simulink model "fcn2A"  (Simulink 7.1)
settings: Solver=VariableStepDiscrete  StartTime=0.0  StopTime=10.0  RelTol=1e-3
undefined symbols (not defined in the file or in its folder): DiscIntNeverNeededParam
settings Model: Creator=W7  LastModifiedBy=W7
settings DataIOCC: ExternalInput=[u]  LoadExternalInput=on
settings DebuggingCC: SolverPrmCheckMsg=none

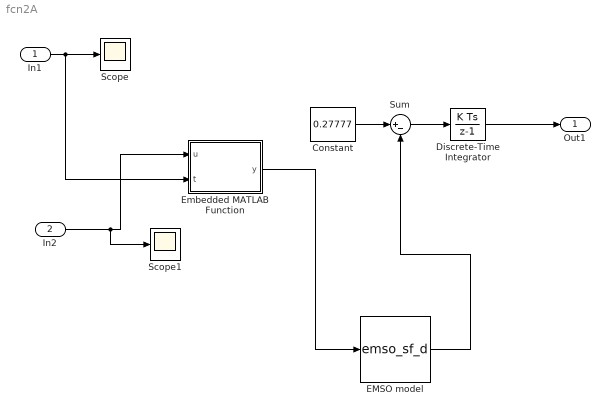
== system fcn2A ==
  In1 : Inport  OutDataType=sfix(16)  OutScaling=2^0
  In2 : Inport  Port=2  OutDataType=sfix(16)  OutScaling=2^0  Interpolate=off
  Constant : Constant  Value=0.27777  OutDataType=sfix(16)  OutScaling=2^0
  Discrete-Time Integrator : DiscreteIntegrator  OutDataType=sfix(16)  OutScaling=2^0  ICPrevOutput=DiscIntNeverNeededParam  ICPrevScaledInput=DiscIntNeverNeededParam
  EMSO model : S-Function  FunctionName=emso_sf_d  Parameters='emso_uotr.ems',1,1,1  EnableBusSupport=off
  Embedded MATLAB Function : Stateflow chart
  Scope : Scope
  Scope1 : Scope
  Sum : Sum  Inputs=|+-  OutDataType=sfix(16)  OutScaling=2^0
  Out1 : Outport
  wires:
  In2/1 -> Embedded MATLAB Function/1(u), Scope1/1
  In1/1 -> Scope/1, Embedded MATLAB Function/2(t)
  EMSO model/1 -> Sum/2
  Embedded MATLAB Function/1(y) -> EMSO model/1
  Discrete-Time Integrator/1 -> Out1/1
  Constant/1 -> Sum/1
  Sum/1 -> Discrete-Time Integrator/1

== matlab function Embedded MATLAB Function ==
  data: u input double; y output double; t input double
function y = fcn(u,t)
% This block supports the Embedded MATLAB subset.
% See the help menu for details. 

    y= u;
end
